simulink model "RobustFormationControl_IntegerModel"  (R2023a)
settings: Solver=ode3  StartTime=0.0  StopTime=30  FixedStep=0.0001  RelTol=1e-3
InitFcn:
  | % % Parameters for the fractional order NTFSMC:
  | % Sliding Surface " Sx, Sy, and Sz ":
  | %------------------------
  | % 10
  | % 10
  | cx = 2*[4 4 4];
  | cxx = 1*[0.01 0.01 0.01];
  | 
  | cx1 = cx(1);
  | cy1 = cx(2);
  | cz1 = cx(3);
  | 
  | cx2 = cxx(1);
  | cy2 = cxx(2);
  | cz2 = cxx(3);
  | 
  | alpha1 = [0.6 0.6 0.6];
  | alpha2 = [0.1 0.1 0.1];
  | 
  | gammaX = [3 3 3];
  | gx  = gammaX(1);
  | gy = gammaX(2);
  | gz = gammaX(3);
  | 
  | p = 10;
  | q = 10;
  | 
  | % Sliding Surface " S_Phi , S_Theta, and  S_Psi":
  | %------------------------
  | cP = 2*[4 4 4];
  | cPP = 1*[0.01 0.01 0.01 0.01];
  | 
  | cPhi1 = cP(1);
  | cTheta1 = cP(2);
  | cPsi1 = cP(3);
  | 
  | cPhi2 = cPP(1);
  | cTheta2 = cPP(2);
  | cPsi2 = cPP(3);
  | gammaP = [3 3 3];
  | 
  | %=========================
  | %=========================
  | SigmaX = 1*[0.01 0.01 0.01];
  | SigmaXX =1*[1 1 1];
  | 
  | Sigma1X = SigmaX(1);
  | Sigma1Y = SigmaX(2);
  | Sigma1Z = SigmaX(3);
  | %-----
  | Sigma2X = SigmaXX(1);
  | Sigma2Y = SigmaXX(2);
  | Sigma2Z = SigmaXX(3);
  | 
  | 
  | SigmaP = 1*[0.01 0.01 0.01];
  | SigmaPP =1*[1 1 1];
  | 
  | Sigma1Phi   = SigmaP(1);
  | Sigma1Theta = SigmaP(2);
  | Sigma1Psi   = SigmaP(3);
  | %----
  | Sigma2Phi   = SigmaPP(1);
  | Sigma2Theta = SigmaPP(2);
  | Sigma2Psi   = SigmaPP(3);
  | 
  | q0 = 0.01;
  | q1 = 0.01;
  | q2 = 0.01;
  | w = 0;
  | %=========================================
  | %=========================================
  | %=========================================
  | %=========================================
  | %=========================================
  | %=========================================
  | %=========================================
  | %=========================================
  | 
  | cxF = 0.01*[4 4 4];
  | cxxF = 1*[0.01 0.01 0.01];
  | 
  | cxF1 = cxF(1);
  | cyF1 = cxF(2);
  | czF1 = cxF(3);
  | 
  | cxF2 = cxxF(1);
  | cyF2 = cxxF(2);
  | czF2 = cxxF(3);
  | 
  | alphaF1 = [0.9 0.9 0.9];
  | alphaF2 = [0.1 0.1 0.1];
  | 
  | gammaX_F = 1.5*[1 1 1];
  | gxF  = gammaX_F(1);
  | gyF = gammaX_F(2);
  | gzF = gammaX_F(3);
  | 
  | % Sliding Surface " S_Phi , S_Theta, and  S_Psi":
  | %------------------------
  | cPF = 1*[4 4 4];
  | cPPF = 1*[0.01 0.01 0.01 0.01];
  | 
  | cPhiF1 = cPF(1);
  | cThetaF1 = cPF(2);
  | cPsiF1 = cPF(3);
  | 
  | cPhiF2 = cPPF(1);
  | cThetaF2 = cPPF(2);
  | cPsiF2 = cPPF(3);
  | gammaP_F = [1 1 1];
  | 
  | %=========================
  | %=========================
  | SigmaXF = 1000*[0.01 0.01 0.01];
  | SigmaXXF =10*[1 1 1];
  | 
  | Sigma1XF = SigmaXF(1);
  | Sigma1YF = SigmaXF(2);
  | Sigma1ZF = SigmaXF(3);
  | %-----
  | Sigma2XF = SigmaXXF(1);
  | Sigma2YF = SigmaXXF(2);
  | Sigma2ZF = SigmaXXF(3);
  | 
  | 
  | SigmaPF = [0.01 0.01 0.01];
  | SigmaPPF =[1 1 1];
  | 
  | Sigma1PhiF   = SigmaPF(1);
  | Sigma1ThetaF = SigmaPF(2);
  | Sigma1PsiF   = SigmaPF(3);
  | %----
  | Sigma2PhiF   = SigmaPPF(1);
  | Sigma2ThetaF = SigmaPPF(2);
  | Sigma2PsiF   = SigmaPPF(3);
  | 
  | % Gain for Exteral Disturbance
  | Dis = 0;
  | dis = 0;
values from neighbouring files (symbols this model uses):
  a1 = (Iyy - Izz)/Ixx    (= -0.812397034596)    [init_quadrotor_params.m]
  a2 = (Izz - Ixx)/Iyy    (= 0.812397034596)    [init_quadrotor_params.m]
  a3 = (Ixx - Iyy)/Izz    (= 0)    [init_quadrotor_params.m]
  a4 = - Ktx/m    (= -0.00114547325103)    [init_quadrotor_params.m]
  a5 = - Kty/m    (= -0.00114547325103)    [init_quadrotor_params.m]
  a6 = - Ktz/m    (= -0.00130740740741)    [init_quadrotor_params.m]
  b = 2.980e-5    (= 2.98e-05)    [init_quadrotor_params.m]
  b1 = - Jr/Ixx    (= -0.00584534596376)    [init_quadrotor_params.m]
  b2 = Jr/Iyy    (= 0.00584534596376)    [init_quadrotor_params.m]
  b3 = - Kfz/Izz    (= -0.0721963413248)    [init_quadrotor_params.m]
  b4 = 1/m    (= 2.05761316872)    [init_quadrotor_params.m]
  b5 = 1/m    (= 2.05761316872)    [init_quadrotor_params.m]
  b6 = 1/m    (= 2.05761316872)    [init_quadrotor_params.m]
  c1 = - Kfx/Ixx    (= -0.114641680395)    [init_quadrotor_params.m]
  c2 = - Kfy/Iyy    (= -0.114641680395)    [init_quadrotor_params.m]
  c3 = 1/Izz    (= 113.62345188)    [init_quadrotor_params.m]
  d = 1.12e-06    [init_quadrotor_params.m]
  d1 = L/Ixx    (= 46.334431631)    [init_quadrotor_params.m]
  d2 = L/Iyy    (= 46.334431631)    [init_quadrotor_params.m]
  g = 9.81    [init_quadrotor_params.m]
  Ixx = 4.856e-3    (= 0.004856)    [init_quadrotor_params.m]
  Iyy = 4.856e-3    (= 0.004856)    [init_quadrotor_params.m]
  Izz = 8.801e-3    (= 0.008801)    [init_quadrotor_params.m]
  Jr = 2.8385e-5    (= 2.8385e-05)    [init_quadrotor_params.m]
  Kfx = 5.567e-4    (= 0.0005567)    [init_quadrotor_params.m]
  Kfy = 5.567e-4    (= 0.0005567)    [init_quadrotor_params.m]
  Kfz = 6.354e-4    (= 0.0006354)    [init_quadrotor_params.m]
  Ktx = 5.5670e-4    (= 0.0005567)    [init_quadrotor_params.m]
  Kty = 5.5670e-4    (= 0.0005567)    [init_quadrotor_params.m]
  Ktz = 6.3540e-4    (= 0.0006354)    [init_quadrotor_params.m]
  L = 0.225    [init_quadrotor_params.m]
  m = 0.486    [init_quadrotor_params.m]
libraries: fod x120, eeStairGenerator x5
(part 1 of 9)
settings Model: Creator=jofan  LastModifiedBy=jofan
settings DataIOCC: ReturnWorkspaceOutputs=off

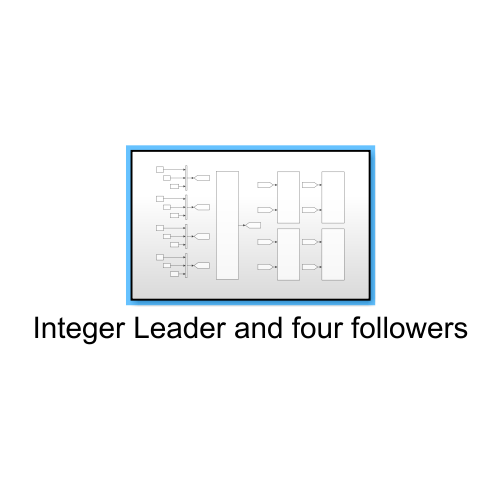
[thumbnail: Simulink's stored preview of the top-level diagram]
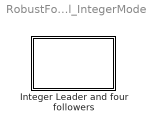
== system RobustFormationControl_IntegerModel ==
  Integer Leader and four followers : Subsystem

== system RobustFormationControl_IntegerModel/Integer Leader and four followers ==
  Follower 1 System : Subsystem
  Follower 2 System : Subsystem
  Follower 3 System : Subsystem
  Follower 4 System : Subsystem
  Leader System : Subsystem
  Mux{,1..3} (4 alike) : Mux  Inputs=3
  dX : Constant  Value=-2
  dX1 : Constant  Value=-2
  dX2 : Constant  Value=-4
  dX3 : Constant  Value=-4
  dY : Constant  Value=2
  dY1 : Constant  Value=-2
  dY2 : Constant  Value=4
  dY3 : Constant  Value=-4
  dZ{,1..3} (4 alike) : Constant  Value=0
  wires:
  dY/1 -> Mux/2
  dZ/1 -> Mux/3
  dX/1 -> Mux/1
  dY1/1 -> Mux1/2
  dZ1/1 -> Mux1/3
  dX1/1 -> Mux1/1
  dX2/1 -> Mux2/1
  dZ2/1 -> Mux2/3
  dY2/1 -> Mux2/2
  dY3/1 -> Mux3/2
  dZ3/1 -> Mux3/3
  dX3/1 -> Mux3/1
  Mux/1 -> [dXYZ]
  Mux1/1 -> [dXYZ1]
  Mux2/1 -> [dXYZ2]
  Mux3/1 -> [dXYZ3]
  Leader System/1(xLeader) -> [xyzL]
  [xyzL] -> Follower 1 System/1(xLeader)
  [xyzL] -> Follower 2 System/1(xLeader)
  [xyzL] -> Follower 4 System/1(xLeader)
  [xyzL] -> Follower 3 System/1(xLeader)
  [dXYZ] -> Follower 1 System/2(dXYZ)
  [dXYZ2] -> Follower 3 System/2(dXYZ)
  [dXYZ1] -> Follower 2 System/2(dXYZ)
  [dXYZ3] -> Follower 4 System/2(dXYZ)

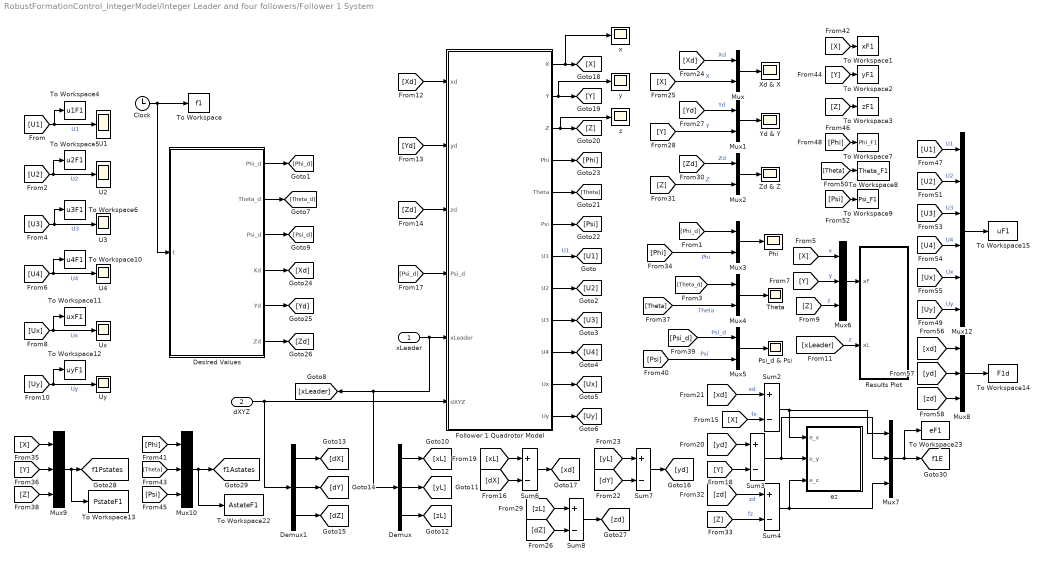
== system RobustFormationControl_IntegerModel/Integer Leader and four followers/Follower 1 System ==
  xLeader : Inport
  dXYZ : Inport  Port=2
  " Phi " : Scope
  Clock : Clock
  Demux : Demux  Outputs=3
  Demux1 : Demux  Outputs=3
  Desired Values : Subsystem
  Follower 1 Quadrotor Model : Subsystem
  Mux{,1..5} (6 alike) : Mux  Inputs=2
  Mux{6..10} (5 alike) : Mux  Inputs=3
  Mux12 : Mux  Inputs=6
  Psi_d & Psi : Scope
  Results Plot : Subsystem
  Sum{2..4,6..8} (6 alike) : Sum  Inputs=+-
  "Theta " : Scope
  To Workspace : ToWorkspace  VariableName=f1  SampleTime=0.03
  To Workspace1 : ToWorkspace  VariableName=xF1  SampleTime=0.03
  To Workspace10 : ToWorkspace  VariableName=u4F1  SampleTime=0.03
  To Workspace11 : ToWorkspace  VariableName=uxF1  SampleTime=0.03
  To Workspace12 : ToWorkspace  VariableName=uyF1  SampleTime=0.03
  To Workspace13 : ToWorkspace  VariableName=PstateF1  SampleTime=-1
  To Workspace14 : ToWorkspace  VariableName=F1d  SampleTime=-1
  To Workspace15 : ToWorkspace  VariableName=uF1  SampleTime=-1
  To Workspace2 : ToWorkspace  VariableName=yF1  SampleTime=0.03
  To Workspace22 : ToWorkspace  VariableName=AstateF1  SampleTime=-1
  To Workspace23 : ToWorkspace  VariableName=eF1  SampleTime=-1
  To Workspace3 : ToWorkspace  VariableName=zF1  SampleTime=0.03
  To Workspace4 : ToWorkspace  VariableName=u1F1  SampleTime=0.03
  To Workspace5 : ToWorkspace  VariableName=u2F1  SampleTime=0.03
  To Workspace6 : ToWorkspace  VariableName=u3F1  SampleTime=0.03
  To Workspace7 : ToWorkspace  VariableName=Phi_F1  SampleTime=0.03
  To Workspace8 : ToWorkspace  VariableName=Theta_F1  SampleTime=0.03
  To Workspace9 : ToWorkspace  VariableName=Psi_F1  SampleTime=0.03
  "U1 " : Scope
  U2 : Scope
  "U3 " : Scope
  "U4 " : Scope
  Ux : Scope
  Uy : Scope
  "Xd & X " : Scope
  Yd & Y : Scope
  "Zd & Z " : Scope
  ez : Subsystem
  x : Scope
  y : Scope
  z : Scope
  tag scope: f1Astates=global, f1E=global, f1Pstates=global
  wires:
  Mux4/1 -> "Theta "/1
  [U2] -> To Workspace5/1, U2/1  "U2"
  [Yd] -> Mux1/1  "Yd"
  Follower 1 Quadrotor Model/10(U4) -> [U4]
  [Zd] -> Follower 1 Quadrotor Model/3(zd)
  [U4] -> To Workspace10/1, "U4 "/1  "U4"
  [Psi] -> To Workspace9/1
  [Z] -> Mux2/2  "Z"
  Follower 1 Quadrotor Model/2(Y) -> y/1, [Y]
  Clock/1 -> To Workspace/1, Desired Values/1(t)
  Follower 1 Quadrotor Model/7(U1) -> [U1]  "U1"
  Desired Values/2(Theta_d) -> [Theta_d]
  Mux2/1 -> "Zd & Z "/1
  [Theta] -> To Workspace8/1
  [Xd] -> Mux/1  "Xd"
  Follower 1 Quadrotor Model/12(Uy) -> [Uy]
  [Y] -> To Workspace2/1
  Follower 1 Quadrotor Model/11(Ux) -> [Ux]
  [X] -> To Workspace1/1
  [Yd] -> Follower 1 Quadrotor Model/2(yd)
  Mux/1 -> "Xd & X "/1
  Follower 1 Quadrotor Model/1(X) -> x/1, [X]
  Mux3/1 -> " Phi "/1
  Follower 1 Quadrotor Model/5(Theta) -> [Theta]
  Mux5/1 -> Psi_d & Psi/1
  [X] -> Mux/2  "X"
  Follower 1 Quadrotor Model/9(U3) -> [U3]
  [Theta] -> Mux4/2  "Theta"
  [Y] -> Mux1/2  "Y"
  [Uy] -> To Workspace12/1, Uy/1  "Uy"
  Desired Values/3(Psi_d) -> [Psi_d]
  Follower 1 Quadrotor Model/3(Z) -> z/1, [Z]
  [U1] -> To Workspace4/1, "U1 "/1  "U1"
  [Ux] -> To Workspace11/1, Ux/1  "Ux"
  Desired Values/6(Zd) -> [Zd]
  [Phi] -> Mux3/2  "Phi"
  Mux1/1 -> Yd & Y/1
  [Xd] -> Follower 1 Quadrotor Model/1(xd)
  [Psi] -> Mux5/2  "Psi"
  [Z] -> To Workspace3/1
  Follower 1 Quadrotor Model/8(U2) -> [U2]
  [Theta_d] -> Mux4/1
  [Psi_d] -> Mux5/1  "Psi_d"
  [Zd] -> Mux2/1  "Zd"
  [U3] -> To Workspace6/1, "U3 "/1  "U3"
  Desired Values/5(Yd) -> [Yd]
  [Psi_d] -> Follower 1 Quadrotor Model/4(Psi_d)
  Follower 1 Quadrotor Model/6(Psi) -> [Psi]
  Follower 1 Quadrotor Model/4(Phi) -> [Phi]
  Desired Values/4(Xd) -> [Xd]
  [Phi_d] -> Mux3/1
  Desired Values/1(Phi_d) -> [Phi_d]
  [Phi] -> To Workspace7/1
  [Z] -> Mux6/3  "z"
  [X] -> Mux6/1  "x"
  [xLeader] -> Results Plot/2(xL)  "z"
  Mux6/1 -> Results Plot/1(xF)
  [Y] -> Mux6/2  "y"
  Sum7/1 -> [yd]
  [dY] -> Sum7/2
  [yL] -> Sum7/1
  Demux/3 -> [zL]
  xLeader/1 -> [xLeader], Demux/1, Follower 1 Quadrotor Model/5(xLeader)
  Demux1/1 -> [dX]
  [zd] -> Sum4/1  "zd"
  Demux/1 -> [xL]
  [X] -> Sum2/2  "fx"
  dXYZ/1 -> Demux1/1, Follower 1 Quadrotor Model/6(dXYZ)
  Demux1/2 -> [dY]
  [xL] -> Sum6/1
  Sum4/1 -> Mux7/3, ez/3(e_z)
  Sum3/1 -> Mux7/2, ez/2(e_y)
  Sum2/1 -> Mux7/1, ez/1(e_x)
  [dZ] -> Sum8/2
  [Z] -> Sum4/2  "fz"
  Demux/2 -> [yL]
  [dX] -> Sum6/2
  [yd] -> Sum3/1
  [Y] -> Sum3/2
  [xd] -> Sum2/1  "xd"
  Sum8/1 -> [zd]
  Demux1/3 -> [dZ]
  [zL] -> Sum8/1
  Sum6/1 -> [xd]
  Mux10/1 -> To Workspace22/1, [f1Astates]
  [Psi] -> Mux10/3
  [Phi] -> Mux10/1
  Mux9/1 -> To Workspace13/1, [f1Pstates]
  [Z] -> Mux9/3
  [Y] -> Mux9/2
  [X] -> Mux9/1
  [Theta] -> Mux10/2
  Mux7/1 -> To Workspace23/1, [f1E]
  [Ux] -> Mux12/5  "Ux"
  [U3] -> Mux12/3  "U3"
  [U2] -> Mux12/2  "U2"
  [U4] -> Mux12/4  "U4"
  [Uy] -> Mux12/6  "Uy"
  [U1] -> Mux12/1  "U1"
  Mux8/1 -> To Workspace14/1
  [xd] -> Mux8/1
  [yd] -> Mux8/2
  [zd] -> Mux8/3
  Mux12/1 -> To Workspace15/1

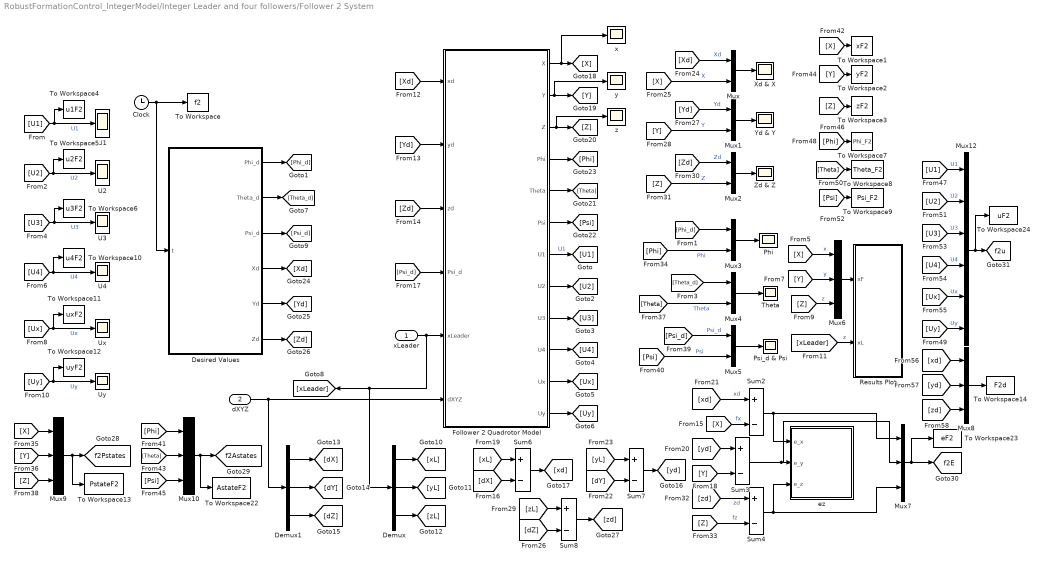
== system RobustFormationControl_IntegerModel/Integer Leader and four followers/Follower 2 System ==
  xLeader : Inport
  dXYZ : Inport  Port=2
  " Phi " : Scope
  Clock : Clock
  Demux : Demux  Outputs=3
  Demux1 : Demux  Outputs=3
  Desired Values : Subsystem
  Follower 2 Quadrotor Model : Subsystem
  Mux{,1..5} (6 alike) : Mux  Inputs=2
  Mux{6..10} (5 alike) : Mux  Inputs=3
  Mux12 : Mux  Inputs=6
  Psi_d & Psi : Scope
  Results Plot : Subsystem
  Sum{2..4,6..8} (6 alike) : Sum  Inputs=+-
  "Theta " : Scope
  To Workspace : ToWorkspace  VariableName=f2  SampleTime=0.03
  To Workspace1 : ToWorkspace  VariableName=xF2  SampleTime=0.03
  To Workspace10 : ToWorkspace  VariableName=u4F2  SampleTime=0.03
  To Workspace11 : ToWorkspace  VariableName=uxF2  SampleTime=0.03
  To Workspace12 : ToWorkspace  VariableName=uyF2  SampleTime=0.03
  To Workspace13 : ToWorkspace  VariableName=PstateF2  SampleTime=-1
  To Workspace14 : ToWorkspace  VariableName=F2d  SampleTime=-1
  To Workspace2 : ToWorkspace  VariableName=yF2  SampleTime=0.03
  To Workspace22 : ToWorkspace  VariableName=AstateF2  SampleTime=-1
  To Workspace23 : ToWorkspace  VariableName=eF2  SampleTime=-1
  To Workspace24 : ToWorkspace  VariableName=uF2  SampleTime=-1
  To Workspace3 : ToWorkspace  VariableName=zF2  SampleTime=0.03
  To Workspace4 : ToWorkspace  VariableName=u1F2  SampleTime=0.03
  To Workspace5 : ToWorkspace  VariableName=u2F2  SampleTime=0.03
  To Workspace6 : ToWorkspace  VariableName=u3F2  SampleTime=0.03
  To Workspace7 : ToWorkspace  VariableName=Phi_F2  SampleTime=0.03
  To Workspace8 : ToWorkspace  VariableName=Theta_F2  SampleTime=0.03
  To Workspace9 : ToWorkspace  VariableName=Psi_F2  SampleTime=0.03
  "U1 " : Scope
  U2 : Scope
  "U3 " : Scope
  "U4 " : Scope
  Ux : Scope
  Uy : Scope
  "Xd & X " : Scope
  Yd & Y : Scope
  "Zd & Z " : Scope
  ez : Subsystem
  x : Scope
  y : Scope
  z : Scope
  tag scope: f2Astates=global, f2E=global, f2Pstates=global, f2u=global
  wires:
  Mux4/1 -> "Theta "/1
  [U2] -> To Workspace5/1, U2/1  "U2"
  [Yd] -> Mux1/1  "Yd"
  Follower 2 Quadrotor Model/10(U4) -> [U4]
  [Zd] -> Follower 2 Quadrotor Model/3(zd)
  [U4] -> To Workspace10/1, "U4 "/1  "U4"
  [Psi] -> To Workspace9/1
  [Z] -> Mux2/2  "Z"
  Follower 2 Quadrotor Model/2(Y) -> y/1, [Y]
  Clock/1 -> To Workspace/1, Desired Values/1(t)
  Follower 2 Quadrotor Model/7(U1) -> [U1]  "U1"
  Desired Values/2(Theta_d) -> [Theta_d]
  Mux2/1 -> "Zd & Z "/1
  [Theta] -> To Workspace8/1
  [Xd] -> Mux/1  "Xd"
  Follower 2 Quadrotor Model/12(Uy) -> [Uy]
  [Y] -> To Workspace2/1
  Follower 2 Quadrotor Model/11(Ux) -> [Ux]
  [X] -> To Workspace1/1
  [Yd] -> Follower 2 Quadrotor Model/2(yd)
  Mux/1 -> "Xd & X "/1
  Follower 2 Quadrotor Model/1(X) -> x/1, [X]
  Mux3/1 -> " Phi "/1
  Follower 2 Quadrotor Model/5(Theta) -> [Theta]
  Mux5/1 -> Psi_d & Psi/1
  [X] -> Mux/2  "X"
  Follower 2 Quadrotor Model/9(U3) -> [U3]
  [Theta] -> Mux4/2  "Theta"
  [Y] -> Mux1/2  "Y"
  [Uy] -> To Workspace12/1, Uy/1  "Uy"
  Desired Values/3(Psi_d) -> [Psi_d]
  Follower 2 Quadrotor Model/3(Z) -> z/1, [Z]
  [U1] -> To Workspace4/1, "U1 "/1  "U1"
  [Ux] -> To Workspace11/1, Ux/1  "Ux"
  Desired Values/6(Zd) -> [Zd]
  [Phi] -> Mux3/2  "Phi"
  Mux1/1 -> Yd & Y/1
  [Xd] -> Follower 2 Quadrotor Model/1(xd)
  [Psi] -> Mux5/2  "Psi"
  [Z] -> To Workspace3/1
  Follower 2 Quadrotor Model/8(U2) -> [U2]
  [Theta_d] -> Mux4/1
  [Psi_d] -> Mux5/1  "Psi_d"
  [Zd] -> Mux2/1  "Zd"
  [U3] -> To Workspace6/1, "U3 "/1  "U3"
  Desired Values/5(Yd) -> [Yd]
  [Psi_d] -> Follower 2 Quadrotor Model/4(Psi_d)
  Follower 2 Quadrotor Model/6(Psi) -> [Psi]
  Follower 2 Quadrotor Model/4(Phi) -> [Phi]
  Desired Values/4(Xd) -> [Xd]
  [Phi_d] -> Mux3/1
  Desired Values/1(Phi_d) -> [Phi_d]
  [Phi] -> To Workspace7/1
  xLeader/1 -> Demux/1, [xLeader], Follower 2 Quadrotor Model/5(xLeader)
  [Z] -> Mux6/3  "z"
  [X] -> Mux6/1  "x"
  [xLeader] -> Results Plot/2(xL)  "z"
  Mux6/1 -> Results Plot/1(xF)
  [Y] -> Mux6/2  "y"
  Sum7/1 -> [yd]
  [dY] -> Sum7/2
  [yL] -> Sum7/1
  Demux/3 -> [zL]
  Demux1/1 -> [dX]
  [zd] -> Sum4/1  "zd"
  Demux/1 -> [xL]
  [X] -> Sum2/2  "fx"
  dXYZ/1 -> Demux1/1, Follower 2 Quadrotor Model/6(dXYZ)
  Demux1/2 -> [dY]
  [xL] -> Sum6/1
  Sum4/1 -> Mux7/3, ez/3(e_z)
  Sum3/1 -> Mux7/2, ez/2(e_y)
  Sum2/1 -> Mux7/1, ez/1(e_x)
  [dZ] -> Sum8/2
  [Z] -> Sum4/2  "fz"
  Demux/2 -> [yL]
  [dX] -> Sum6/2
  [yd] -> Sum3/1
  [Y] -> Sum3/2
  [xd] -> Sum2/1  "xd"
  Sum8/1 -> [zd]
  Demux1/3 -> [dZ]
  [zL] -> Sum8/1
  Sum6/1 -> [xd]
  [X] -> Mux9/1
  [Psi] -> Mux10/3
  [Theta] -> Mux10/2
  Mux9/1 -> To Workspace13/1, [f2Pstates]
  [Y] -> Mux9/2
  [Phi] -> Mux10/1
  Mux10/1 -> To Workspace22/1, [f2Astates]
  [Z] -> Mux9/3
  Mux7/1 -> To Workspace23/1, [f2E]
  [U3] -> Mux12/3  "U3"
  [Ux] -> Mux12/5  "Ux"
  Mux12/1 -> To Workspace24/1, [f2u]
  [Uy] -> Mux12/6  "Uy"
  [U4] -> Mux12/4  "U4"
  [U2] -> Mux12/2  "U2"
  [U1] -> Mux12/1  "U1"
  Mux8/1 -> To Workspace14/1
  [zd] -> Mux8/3
  [xd] -> Mux8/1
  [yd] -> Mux8/2

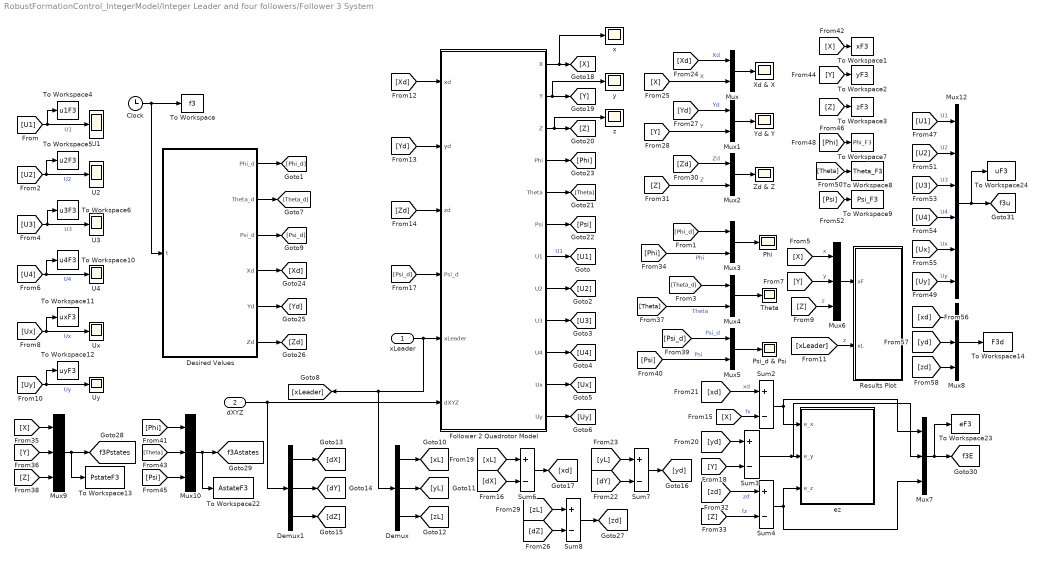
== system RobustFormationControl_IntegerModel/Integer Leader and four followers/Follower 3 System ==
  xLeader : Inport
  dXYZ : Inport  Port=2
  " Phi " : Scope
  Clock : Clock
  Demux : Demux  Outputs=3
  Demux1 : Demux  Outputs=3
  Desired Values : Subsystem
  Follower 2 Quadrotor Model : Subsystem
  Mux{,1..5} (6 alike) : Mux  Inputs=2
  Mux{6..10} (5 alike) : Mux  Inputs=3
  Mux12 : Mux  Inputs=6
  Psi_d & Psi : Scope
  Results Plot : Subsystem
  Sum{2..4,6..8} (6 alike) : Sum  Inputs=+-
  "Theta " : Scope
  To Workspace : ToWorkspace  VariableName=f3  SampleTime=0.03
  To Workspace1 : ToWorkspace  VariableName=xF3  SampleTime=0.03
  To Workspace10 : ToWorkspace  VariableName=u4F3  SampleTime=0.03
  To Workspace11 : ToWorkspace  VariableName=uxF3  SampleTime=0.03
  To Workspace12 : ToWorkspace  VariableName=uyF3  SampleTime=0.03
  To Workspace13 : ToWorkspace  VariableName=PstateF3  SampleTime=-1
  To Workspace14 : ToWorkspace  VariableName=F3d  SampleTime=-1
  To Workspace2 : ToWorkspace  VariableName=yF3  SampleTime=0.03
  To Workspace22 : ToWorkspace  VariableName=AstateF3  SampleTime=-1
  To Workspace23 : ToWorkspace  VariableName=eF3  SampleTime=-1
  To Workspace24 : ToWorkspace  VariableName=uF3  SampleTime=-1
  To Workspace3 : ToWorkspace  VariableName=zF3  SampleTime=0.03
  To Workspace4 : ToWorkspace  VariableName=u1F3  SampleTime=0.03
  To Workspace5 : ToWorkspace  VariableName=u2F3  SampleTime=0.03
  To Workspace6 : ToWorkspace  VariableName=u3F3  SampleTime=0.03
  To Workspace7 : ToWorkspace  VariableName=Phi_F3  SampleTime=0.03
  To Workspace8 : ToWorkspace  VariableName=Theta_F3  SampleTime=0.03
  To Workspace9 : ToWorkspace  VariableName=Psi_F3  SampleTime=0.03
  "U1 " : Scope
  U2 : Scope
  "U3 " : Scope
  "U4 " : Scope
  Ux : Scope
  Uy : Scope
  "Xd & X " : Scope
  Yd & Y : Scope
  "Zd & Z " : Scope
  ez : Subsystem
  x : Scope
  y : Scope
  z : Scope
  tag scope: f3Astates=global, f3E=global, f3Pstates=global, f3u=global
  wires:
  [Y] -> Mux6/2  "y"
  Mux6/1 -> Results Plot/1(xF)
  [xLeader] -> Results Plot/2(xL)  "z"
  [X] -> Mux6/1  "x"
  [Z] -> Mux6/3  "z"
  xLeader/1 -> Follower 2 Quadrotor Model/5(xLeader), Demux/1, [xLeader]
  [Phi] -> To Workspace7/1
  Desired Values/1(Phi_d) -> [Phi_d]
  [Phi_d] -> Mux3/1
  Desired Values/4(Xd) -> [Xd]
  Follower 2 Quadrotor Model/4(Phi) -> [Phi]
  Follower 2 Quadrotor Model/6(Psi) -> [Psi]
  [Psi_d] -> Follower 2 Quadrotor Model/4(Psi_d)
  Desired Values/5(Yd) -> [Yd]
  [U3] -> "U3 "/1, To Workspace6/1  "U3"
  [Zd] -> Mux2/1  "Zd"
  [Psi_d] -> Mux5/1  "Psi_d"
  [Theta_d] -> Mux4/1
  Follower 2 Quadrotor Model/8(U2) -> [U2]
  [Z] -> To Workspace3/1
  [Psi] -> Mux5/2  "Psi"
  [Xd] -> Follower 2 Quadrotor Model/1(xd)
  Mux1/1 -> Yd & Y/1
  [Phi] -> Mux3/2  "Phi"
  Desired Values/6(Zd) -> [Zd]
  [Ux] -> Ux/1, To Workspace11/1  "Ux"
  [U1] -> "U1 "/1, To Workspace4/1  "U1"
  Follower 2 Quadrotor Model/3(Z) -> [Z], z/1
  Desired Values/3(Psi_d) -> [Psi_d]
  [Uy] -> Uy/1, To Workspace12/1  "Uy"
  [Y] -> Mux1/2  "Y"
  [Theta] -> Mux4/2  "Theta"
  Follower 2 Quadrotor Model/9(U3) -> [U3]
  [X] -> Mux/2  "X"
  Mux5/1 -> Psi_d & Psi/1
  Follower 2 Quadrotor Model/5(Theta) -> [Theta]
  Mux3/1 -> " Phi "/1
  Follower 2 Quadrotor Model/1(X) -> [X], x/1
  Mux/1 -> "Xd & X "/1
  [Yd] -> Follower 2 Quadrotor Model/2(yd)
  [X] -> To Workspace1/1
  Follower 2 Quadrotor Model/11(Ux) -> [Ux]
  [Y] -> To Workspace2/1
  Follower 2 Quadrotor Model/12(Uy) -> [Uy]
  [Xd] -> Mux/1  "Xd"
  [Theta] -> To Workspace8/1
  Mux2/1 -> "Zd & Z "/1
  Desired Values/2(Theta_d) -> [Theta_d]
  Follower 2 Quadrotor Model/7(U1) -> [U1]  "U1"
  Clock/1 -> Desired Values/1(t), To Workspace/1
  Follower 2 Quadrotor Model/2(Y) -> [Y], y/1
  [Z] -> Mux2/2  "Z"
  [Psi] -> To Workspace9/1
  [U4] -> "U4 "/1, To Workspace10/1  "U4"
  [Zd] -> Follower 2 Quadrotor Model/3(zd)
  Follower 2 Quadrotor Model/10(U4) -> [U4]
  [Yd] -> Mux1/1  "Yd"
  [U2] -> U2/1, To Workspace5/1  "U2"
  Mux4/1 -> "Theta "/1
  Sum7/1 -> [yd]
  [dY] -> Sum7/2
  [yL] -> Sum7/1
  Demux/3 -> [zL]
  Demux1/1 -> [dX]
  [zd] -> Sum4/1  "zd"
  Demux/1 -> [xL]
  [X] -> Sum2/2  "fx"
  dXYZ/1 -> Demux1/1, Follower 2 Quadrotor Model/6(dXYZ)
  Demux1/2 -> [dY]
  [xL] -> Sum6/1
  Sum4/1 -> Mux7/3, ez/3(e_z)
  Sum3/1 -> Mux7/2, ez/2(e_y)
  Sum2/1 -> Mux7/1, ez/1(e_x)
  [dZ] -> Sum8/2
  [Z] -> Sum4/2  "fz"
  Demux/2 -> [yL]
  [dX] -> Sum6/2
  [yd] -> Sum3/1
  [Y] -> Sum3/2
  [xd] -> Sum2/1  "xd"
  Sum8/1 -> [zd]
  Demux1/3 -> [dZ]
  [zL] -> Sum8/1
  Sum6/1 -> [xd]
  [X] -> Mux9/1
  [Psi] -> Mux10/3
  [Theta] -> Mux10/2
  Mux9/1 -> To Workspace13/1, [f3Pstates]
  [Y] -> Mux9/2
  [Phi] -> Mux10/1
  Mux10/1 -> To Workspace22/1, [f3Astates]
  [Z] -> Mux9/3
  Mux7/1 -> To Workspace23/1, [f3E]
  [U3] -> Mux12/3  "U3"
  [Ux] -> Mux12/5  "Ux"
  Mux12/1 -> To Workspace24/1, [f3u]
  [Uy] -> Mux12/6  "Uy"
  [U4] -> Mux12/4  "U4"
  [U2] -> Mux12/2  "U2"
  [U1] -> Mux12/1  "U1"
  Mux8/1 -> To Workspace14/1
  [zd] -> Mux8/3
  [xd] -> Mux8/1
  [yd] -> Mux8/2

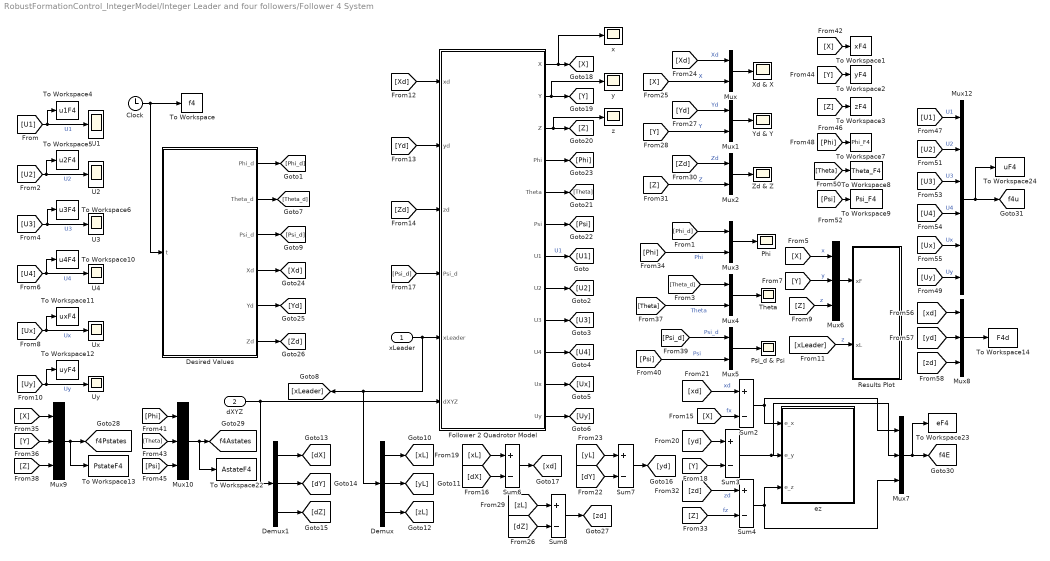
== system RobustFormationControl_IntegerModel/Integer Leader and four followers/Follower 4 System ==
  xLeader : Inport
  dXYZ : Inport  Port=2
  " Phi " : Scope
  Clock : Clock
  Demux : Demux  Outputs=3
  Demux1 : Demux  Outputs=3
  Desired Values : Subsystem
  Follower 2 Quadrotor Model : Subsystem
  Mux{,1..5} (6 alike) : Mux  Inputs=2
  Mux{6..10} (5 alike) : Mux  Inputs=3
  Mux12 : Mux  Inputs=6
  Psi_d & Psi : Scope
  Results Plot : Subsystem
  Sum{2..4,6..8} (6 alike) : Sum  Inputs=+-
  "Theta " : Scope
  To Workspace : ToWorkspace  VariableName=f4  SampleTime=0.03
  To Workspace1 : ToWorkspace  VariableName=xF4  SampleTime=0.03
  To Workspace10 : ToWorkspace  VariableName=u4F4  SampleTime=0.03
  To Workspace11 : ToWorkspace  VariableName=uxF4  SampleTime=0.03
  To Workspace12 : ToWorkspace  VariableName=uyF4  SampleTime=0.03
  To Workspace13 : ToWorkspace  VariableName=PstateF4  SampleTime=-1
  To Workspace14 : ToWorkspace  VariableName=F4d  SampleTime=-1
  To Workspace2 : ToWorkspace  VariableName=yF4  SampleTime=0.03
  To Workspace22 : ToWorkspace  VariableName=AstateF4  SampleTime=-1
  To Workspace23 : ToWorkspace  VariableName=eF4  SampleTime=-1
  To Workspace24 : ToWorkspace  VariableName=uF4  SampleTime=-1
  To Workspace3 : ToWorkspace  VariableName=zF4  SampleTime=0.03
  To Workspace4 : ToWorkspace  VariableName=u1F4  SampleTime=0.03
  To Workspace5 : ToWorkspace  VariableName=u2F4  SampleTime=0.03
  To Workspace6 : ToWorkspace  VariableName=u3F4  SampleTime=0.03
  To Workspace7 : ToWorkspace  VariableName=Phi_F4  SampleTime=0.03
  To Workspace8 : ToWorkspace  VariableName=Theta_F4  SampleTime=0.03
  To Workspace9 : ToWorkspace  VariableName=Psi_F4  SampleTime=0.03
  "U1 " : Scope
  U2 : Scope
  "U3 " : Scope
  "U4 " : Scope
  Ux : Scope
  Uy : Scope
  "Xd & X " : Scope
  Yd & Y : Scope
  "Zd & Z " : Scope
  ez : Subsystem
  x : Scope
  y : Scope
  z : Scope
  tag scope: f4Astates=global, f4E=global, f4Pstates=global, f4u=global
  wires:
  Mux4/1 -> "Theta "/1
  [U2] -> To Workspace5/1, U2/1  "U2"
  [Yd] -> Mux1/1  "Yd"
  Follower 2 Quadrotor Model/10(U4) -> [U4]
  [Zd] -> Follower 2 Quadrotor Model/3(zd)
  [U4] -> To Workspace10/1, "U4 "/1  "U4"
  [Psi] -> To Workspace9/1
  [Z] -> Mux2/2  "Z"
  Follower 2 Quadrotor Model/2(Y) -> y/1, [Y]
  Clock/1 -> To Workspace/1, Desired Values/1(t)
  Follower 2 Quadrotor Model/7(U1) -> [U1]  "U1"
  Desired Values/2(Theta_d) -> [Theta_d]
  Mux2/1 -> "Zd & Z "/1
  [Theta] -> To Workspace8/1
  [Xd] -> Mux/1  "Xd"
  Follower 2 Quadrotor Model/12(Uy) -> [Uy]
  [Y] -> To Workspace2/1
  Follower 2 Quadrotor Model/11(Ux) -> [Ux]
  [X] -> To Workspace1/1
  [Yd] -> Follower 2 Quadrotor Model/2(yd)
  Mux/1 -> "Xd & X "/1
  Follower 2 Quadrotor Model/1(X) -> x/1, [X]
  Mux3/1 -> " Phi "/1
  Follower 2 Quadrotor Model/5(Theta) -> [Theta]
  Mux5/1 -> Psi_d & Psi/1
  [X] -> Mux/2  "X"
  Follower 2 Quadrotor Model/9(U3) -> [U3]
  [Theta] -> Mux4/2  "Theta"
  [Y] -> Mux1/2  "Y"
  [Uy] -> To Workspace12/1, Uy/1  "Uy"
  Desired Values/3(Psi_d) -> [Psi_d]
  Follower 2 Quadrotor Model/3(Z) -> z/1, [Z]
  [U1] -> To Workspace4/1, "U1 "/1  "U1"
  [Ux] -> To Workspace11/1, Ux/1  "Ux"
  Desired Values/6(Zd) -> [Zd]
  [Phi] -> Mux3/2  "Phi"
  Mux1/1 -> Yd & Y/1
  [Xd] -> Follower 2 Quadrotor Model/1(xd)
  [Psi] -> Mux5/2  "Psi"
  [Z] -> To Workspace3/1
  Follower 2 Quadrotor Model/8(U2) -> [U2]
  [Theta_d] -> Mux4/1
  [Psi_d] -> Mux5/1  "Psi_d"
  [Zd] -> Mux2/1  "Zd"
  [U3] -> To Workspace6/1, "U3 "/1  "U3"
  Desired Values/5(Yd) -> [Yd]
  [Psi_d] -> Follower 2 Quadrotor Model/4(Psi_d)
  Follower 2 Quadrotor Model/6(Psi) -> [Psi]
  Follower 2 Quadrotor Model/4(Phi) -> [Phi]
  Desired Values/4(Xd) -> [Xd]
  [Phi_d] -> Mux3/1
  Desired Values/1(Phi_d) -> [Phi_d]
  [Phi] -> To Workspace7/1
  [Z] -> Mux6/3  "z"
  [X] -> Mux6/1  "x"
  [xLeader] -> Results Plot/2(xL)  "z"
  Mux6/1 -> Results Plot/1(xF)
  [Y] -> Mux6/2  "y"
  Sum7/1 -> [yd]
  [dY] -> Sum7/2
  [yL] -> Sum7/1
  Demux/3 -> [zL]
  xLeader/1 -> Demux/1, [xLeader], Follower 2 Quadrotor Model/5(xLeader)
  Demux1/1 -> [dX]
  [zd] -> Sum4/1  "zd"
  Demux/1 -> [xL]
  [X] -> Sum2/2  "fx"
  dXYZ/1 -> Follower 2 Quadrotor Model/6(dXYZ), Demux1/1
  Demux1/2 -> [dY]
  [xL] -> Sum6/1
  Sum4/1 -> Mux7/3, ez/3(e_z)
  Sum3/1 -> Mux7/2, ez/2(e_y)
  Sum2/1 -> Mux7/1, ez/1(e_x)
  [dZ] -> Sum8/2
  [Z] -> Sum4/2  "fz"
  Demux/2 -> [yL]
  [dX] -> Sum6/2
  [yd] -> Sum3/1
  [Y] -> Sum3/2
  [xd] -> Sum2/1  "xd"
  Sum8/1 -> [zd]
  Demux1/3 -> [dZ]
  [zL] -> Sum8/1
  Sum6/1 -> [xd]
  [X] -> Mux9/1
  [Psi] -> Mux10/3
  [Theta] -> Mux10/2
  Mux9/1 -> To Workspace13/1, [f4Pstates]
  [Y] -> Mux9/2
  [Phi] -> Mux10/1
  Mux10/1 -> To Workspace22/1, [f4Astates]
  [Z] -> Mux9/3
  Mux7/1 -> To Workspace23/1, [f4E]
  [U3] -> Mux12/3  "U3"
  [Ux] -> Mux12/5  "Ux"
  Mux12/1 -> To Workspace24/1, [f4u]
  [Uy] -> Mux12/6  "Uy"
  [U4] -> Mux12/4  "U4"
  [U2] -> Mux12/2  "U2"
  [U1] -> Mux12/1  "U1"
  Mux8/1 -> To Workspace14/1
  [zd] -> Mux8/3
  [xd] -> Mux8/1
  [yd] -> Mux8/2

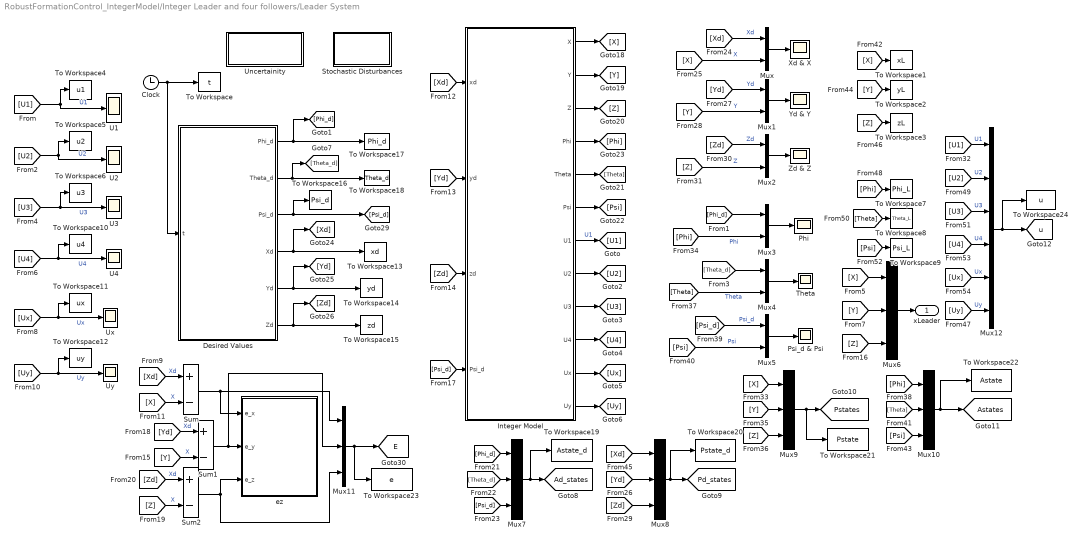
== system RobustFormationControl_IntegerModel/Integer Leader and four followers/Leader System ==
  " Phi " : Scope
  Clock : Clock
  Desired Values : Subsystem
  Integer Model : Subsystem
  Mux{,1..5} (6 alike) : Mux  Inputs=2
  Mux{6..11} (6 alike) : Mux  Inputs=3
  Mux12 : Mux  Inputs=6
  Psi_d & Psi : Scope
  Stochastic Disturbances : Subsystem
  Sum : Sum  Inputs=+-
  Sum1 : Sum  Inputs=+-
  Sum2 : Sum  Inputs=+-
  "Theta " : Scope
  To Workspace : ToWorkspace  VariableName=t  SampleTime=0.03
  To Workspace1 : ToWorkspace  VariableName=xL  SampleTime=0.03
  To Workspace10 : ToWorkspace  VariableName=u4  SampleTime=-1
  To Workspace11 : ToWorkspace  VariableName=ux  SampleTime=0.03
  To Workspace12 : ToWorkspace  VariableName=uy  SampleTime=0.03
  To Workspace13 : ToWorkspace  VariableName=xd  SampleTime=0.03
  To Workspace14 : ToWorkspace  VariableName=yd  SampleTime=0.03
  To Workspace15 : ToWorkspace  VariableName=zd  SampleTime=0.03
  To Workspace16 : ToWorkspace  VariableName=Psi_d  SampleTime=0.03
  To Workspace17 : ToWorkspace  VariableName=Phi_d  SampleTime=0.03
  To Workspace18 : ToWorkspace  VariableName=Theta_d  SampleTime=0.03
  To Workspace19 : ToWorkspace  VariableName=Astate_d  SampleTime=-1
  To Workspace2 : ToWorkspace  VariableName=yL  SampleTime=0.03
  To Workspace20 : ToWorkspace  VariableName=Pstate_d  SampleTime=-1
  To Workspace21 : ToWorkspace  VariableName=Pstate  SampleTime=-1
  To Workspace22 : ToWorkspace  VariableName=Astate  SampleTime=-1
  To Workspace23 : ToWorkspace  VariableName=e  SampleTime=-1
  To Workspace24 : ToWorkspace  VariableName=u  SampleTime=-1
  To Workspace3 : ToWorkspace  VariableName=zL  SampleTime=0.03
  To Workspace4 : ToWorkspace  VariableName=u1  SampleTime=0.03
  To Workspace5 : ToWorkspace  VariableName=u2  SampleTime=0.03
  To Workspace6 : ToWorkspace  VariableName=u3  SampleTime=0.03
  To Workspace7 : ToWorkspace  VariableName=Phi_L  SampleTime=0.03
  To Workspace8 : ToWorkspace  VariableName=Theta_L  SampleTime=0.03
  To Workspace9 : ToWorkspace  VariableName=Psi_L  SampleTime=0.03
  "U1 " : Scope
  U2 : Scope
  "U3 " : Scope
  "U4 " : Scope
  Uncertainity : Subsystem
  Ux : Scope
  Uy : Scope
  "Xd & X " : Scope
  Yd & Y : Scope
  "Zd & Z " : Scope
  ez : Subsystem
  xLeader : Outport
  tag scope: Ad_states=global, Astates=global, E=global, Pd_states=global, Pstates=global, u=global
  wires:
  Mux4/1 -> "Theta "/1
  [U2] -> To Workspace5/1, U2/1  "U2"
  [Yd] -> Mux1/1  "Yd"
  Integer Model/10(U4) -> [U4]
  [Zd] -> Integer Model/3(zd)
  [U4] -> To Workspace10/1, "U4 "/1  "U4"
  [Psi] -> To Workspace9/1
  [Z] -> Mux2/2  "Z"
  Integer Model/2(Y) -> [Y]
  Clock/1 -> To Workspace/1, Desired Values/1(t)
  Integer Model/7(U1) -> [U1]  "U1"
  Desired Values/2(Theta_d) -> To Workspace18/1, [Theta_d]
  Mux2/1 -> "Zd & Z "/1
  [Theta] -> To Workspace8/1
  [Xd] -> Mux/1  "Xd"
  Integer Model/12(Uy) -> [Uy]
  [Y] -> To Workspace2/1
  Integer Model/11(Ux) -> [Ux]
  [X] -> To Workspace1/1
  [Yd] -> Integer Model/2(yd)
  Mux/1 -> "Xd & X "/1
  Integer Model/1(X) -> [X]
  Mux3/1 -> " Phi "/1
  Integer Model/5(Theta) -> [Theta]
  Mux5/1 -> Psi_d & Psi/1
  [X] -> Mux/2  "X"
  Integer Model/9(U3) -> [U3]
  [Theta] -> Mux4/2  "Theta"
  [Y] -> Mux1/2  "Y"
  [Uy] -> To Workspace12/1, Uy/1  "Uy"
  Desired Values/3(Psi_d) -> To Workspace16/1, [Psi_d]
  Integer Model/3(Z) -> [Z]
  [U1] -> To Workspace4/1, "U1 "/1  "U1"
  [Ux] -> To Workspace11/1, Ux/1  "Ux"
  Desired Values/6(Zd) -> [Zd], To Workspace15/1
  [Phi] -> Mux3/2  "Phi"
  Mux1/1 -> Yd & Y/1
  [Xd] -> Integer Model/1(xd)
  [Psi] -> Mux5/2  "Psi"
  [Z] -> To Workspace3/1
  Integer Model/8(U2) -> [U2]
  [Theta_d] -> Mux4/1
  [Psi_d] -> Mux5/1  "Psi_d"
  [Zd] -> Mux2/1  "Zd"
  [U3] -> To Workspace6/1, "U3 "/1  "U3"
  Desired Values/5(Yd) -> [Yd], To Workspace14/1
  [Psi_d] -> Integer Model/4(Psi_d)
  Integer Model/6(Psi) -> [Psi]
  Integer Model/4(Phi) -> [Phi]
  Desired Values/4(Xd) -> [Xd], To Workspace13/1
  [Phi_d] -> Mux3/1
  Desired Values/1(Phi_d) -> To Workspace17/1, [Phi_d]
  [Phi] -> To Workspace7/1
  [X] -> Mux6/1
  Mux6/1 -> xLeader/1
  [Z] -> Mux6/3
  [Y] -> Mux6/2
  [Xd] -> Sum/1  "Xd"
  [X] -> Sum/2  "X"
  [Y] -> Sum1/2  "X"
  [Yd] -> Sum1/1  "Xd"
  [Z] -> Sum2/2  "X"
  [Zd] -> Sum2/1  "Xd"
  Sum1/1 -> Mux11/2, ez/2(e_y)
  Sum/1 -> Mux11/1, ez/1(e_x)
  Sum2/1 -> Mux11/3, ez/3(e_z)
  [Phi_d] -> Mux7/1
  [Theta_d] -> Mux7/2
  [Psi_d] -> Mux7/3
  Mux7/1 -> To Workspace19/1, [Ad_states]
  Mux8/1 -> To Workspace20/1, [Pd_states]
  [Xd] -> Mux8/1
  [Zd] -> Mux8/3
  [Yd] -> Mux8/2
  Mux9/1 -> To Workspace21/1, [Pstates]
  Mux10/1 -> To Workspace22/1, [Astates]
  [Psi] -> Mux10/3
  [Theta] -> Mux10/2
  [X] -> Mux9/1
  [Phi] -> Mux10/1
  [Z] -> Mux9/3
  [Y] -> Mux9/2
  Mux11/1 -> To Workspace23/1, [E]
  Mux12/1 -> To Workspace24/1, [u]
  [U1] -> Mux12/1  "U1"
  [U2] -> Mux12/2  "U2"
  [U3] -> Mux12/3  "U3"
  [U4] -> Mux12/4  "U4"
  [Ux] -> Mux12/5  "Ux"
  [Uy] -> Mux12/6  "Uy"

== system RobustFormationControl_IntegerModel/Integer Leader and four followers/Follower 1 System/Desired Values ==
  t : Inport
  Helical Trajectry : Subsystem  Commented=on
  Helical Trajectry1 : Subsystem
  Step : Step  Time=0  After=0.001  SampleTime=0
  Step Inputs Trajectry : Subsystem  Commented=on
  Phi_d : Outport  VectorParamsAs1DForOutWhenUnconnected=off
  Theta_d : Outport  Port=2  VectorParamsAs1DForOutWhenUnconnected=off
  Psi_d : Outport  Port=3  VectorParamsAs1DForOutWhenUnconnected=off
  Xd : Outport  Port=4  VectorParamsAs1DForOutWhenUnconnected=off
  Yd : Outport  Port=5  VectorParamsAs1DForOutWhenUnconnected=off
  Zd : Outport  Port=6  VectorParamsAs1DForOutWhenUnconnected=off
  wires:
  t/1 -> Helical Trajectry1/1(t), Helical Trajectry/1(t)
  Step/1 -> Theta_d/1, Phi_d/1
  Helical Trajectry1/1(xd) -> Xd/1
  Helical Trajectry1/4(Psi_d) -> Psi_d/1
  Helical Trajectry1/2(yd) -> Yd/1
  Helical Trajectry1/3(zd) -> Zd/1

== system RobustFormationControl_IntegerModel/Integer Leader and four followers/Follower 1 System/Follower 1 Quadrotor Model ==
  xd : Inport
  yd : Inport  Port=2
  zd : Inport  Port=3
  Psi_d : Inport  Port=4
  xLeader : Inport  Port=5
  dXYZ : Inport  Port=6
  Control Module1 : Subsystem
  Quadrotor Dynamic System : Subsystem
  X : Outport  VectorParamsAs1DForOutWhenUnconnected=off
  Y : Outport  Port=2  VectorParamsAs1DForOutWhenUnconnected=off
  Z : Outport  Port=3  VectorParamsAs1DForOutWhenUnconnected=off
  Phi : Outport  Port=4  VectorParamsAs1DForOutWhenUnconnected=off
  Theta : Outport  Port=5  VectorParamsAs1DForOutWhenUnconnected=off
  Psi : Outport  Port=6  VectorParamsAs1DForOutWhenUnconnected=off
  U1 : Outport  Port=7  VectorParamsAs1DForOutWhenUnconnected=off
  U2 : Outport  Port=8  VectorParamsAs1DForOutWhenUnconnected=off
  U3 : Outport  Port=9  VectorParamsAs1DForOutWhenUnconnected=off
  U4 : Outport  Port=10  VectorParamsAs1DForOutWhenUnconnected=off
  Ux : Outport  Port=11  VectorParamsAs1DForOutWhenUnconnected=off
  Uy : Outport  Port=12  VectorParamsAs1DForOutWhenUnconnected=off
  wires:
  Control Module1/5(Ux) -> Ux/1, Quadrotor Dynamic System/5(Ux)  "Ux"
  Quadrotor Dynamic System/2(y = x9) -> [x9], Y/1  "Y"
  Quadrotor Dynamic System/6(Psi) -> [x5], Psi/1  "Psi"
  Control Module1/4(U4) -> U4/1, Quadrotor Dynamic System/4(U4)  "U4"
  Quadrotor Dynamic System/3(z = x11) -> [x11], Z/1  "Z"
  Quadrotor Dynamic System/4(Phi) -> [x1], Phi/1  "Phi"
  Quadrotor Dynamic System/5(Theta) -> [x3], Theta/1  "Theta"
  Quadrotor Dynamic System/1(x = x7) -> [x7], X/1  "X"
  Control Module1/6(Uy) -> Uy/1, Quadrotor Dynamic System/6(Uy)  "Uy"
  Control Module1/1(U1) -> Quadrotor Dynamic System/1(U1), U1/1  "U1"
  Control Module1/2(U2) -> Quadrotor Dynamic System/2(U2), U2/1  "U2"
  Control Module1/3(U3) -> U3/1, Quadrotor Dynamic System/3(U3)  "U3"
  Control Module1/7(Omega) -> Quadrotor Dynamic System/7(Omega)
  Quadrotor Dynamic System/7(x2) -> [x2]
  Quadrotor Dynamic System/12(zdot = x12) -> [x12]
  Quadrotor Dynamic System/11(ydot = x10) -> [x10]
  Quadrotor Dynamic System/10(xdot = x8) -> [x8]
  Quadrotor Dynamic System/9(x6) -> [x6]
  Quadrotor Dynamic System/8(x4) -> [x4]
  [x1] -> Control Module1/1(x1)
  [x2] -> Control Module1/2(x2)
  [x3] -> Control Module1/3(x3)
  [x4] -> Control Module1/4(x4)
  [x5] -> Control Module1/5(x5)
  [x6] -> Control Module1/6(x6)
  [x7] -> Control Module1/7(x7)
  [x8] -> Control Module1/8(x8)
  [x9] -> Control Module1/9(x9)
  [x10] -> Control Module1/10(x10)
  [x11] -> Control Module1/11(x11)
  [x12] -> Control Module1/12(x12)
  xd/1 -> Control Module1/14(" xd")
  yd/1 -> Control Module1/15(yd)
  zd/1 -> Control Module1/16(" zd")
  Psi_d/1 -> Control Module1/13(Psi_d)
  xLeader/1 -> Control Module1/17(xLeader)
  dXYZ/1 -> Control Module1/18(Distance_d)

== system RobustFormationControl_IntegerModel/Integer Leader and four followers/Follower 1 System/Results Plot ==
  note: yL
  xF : Inport
  xL : Inport  Port=2
  Demux : Demux  Outputs=3
  Demux1 : Demux  Outputs=3
  x : Scope  NumInputPorts=2
  y : Scope  NumInputPorts=2
  z : Scope  NumInputPorts=2
  wires:
  xF/1 -> Demux/1
  xL/1 -> Demux1/1
  Demux/1 -> x/1  "xF"
  Demux1/1 -> x/2  "xL"
  Demux/2 -> y/1  "yF"
  Demux1/2 -> y/2
  Demux/3 -> z/1  "zF"
  Demux1/3 -> z/2  "zL"

== system RobustFormationControl_IntegerModel/Integer Leader and four followers/Follower 1 System/ez ==
  note: error analysis for x - position
  note: error analysis for z - position
  note: error analysis for y - position
  e_x : Inport
  e_y : Inport  Port=2
  e_z : Inport  Port=3
  Abs : Abs  SaturateOnIntegerOverflow=off
  Abs1 : Abs  SaturateOnIntegerOverflow=off
  Abs2 : Abs  SaturateOnIntegerOverflow=off
  Clock1 : Clock
  IAE : Display
  IAE1 : Display
  IAE2 : Display
  ISE : Display
  ISE1 : Display
  ISE2 : Display
  ITAE : Display
  ITAE1 : Display
  ITAE2 : Display
  ITSE : Display
  ITSE1 : Display
  ITSE2 : Display
  Integrator{,1..11} (12 alike) : Integrator
  Math Function : Math  Operator=square
  Math Function1 : Math  Operator=square
  Math Function2 : Math  Operator=square
  Mux : Mux
  Mux1 : Mux
  Mux2 : Mux
  Product{,1..5} (6 alike) : Product
  To Workspace : ToWorkspace  VariableName=Ex1  SampleTime=-1
  To Workspace1 : ToWorkspace  VariableName=Ez1  SampleTime=-1
  To Workspace2 : ToWorkspace  VariableName=Ey1  SampleTime=-1
  wires:
  Abs/1 -> Product/1, Integrator/1
  Integrator/1 -> Mux/1, IAE/1
  Math Function/1 -> Product1/1, Integrator1/1
  Integrator1/1 -> Mux/2, ISE/1
  Product/1 -> Integrator2/1
  Integrator2/1 -> Mux/3, ITAE/1
  Product1/1 -> Integrator3/1
  Integrator3/1 -> Mux/4, ITSE/1
  [time] -> Product1/2, Product/2
  [time] -> Product2/2, Product3/2
  Integrator7/1 -> Mux2/4, ITSE1/1
  Product3/1 -> Integrator7/1
  Integrator6/1 -> Mux2/3, ITAE1/1
  Product2/1 -> Integrator6/1
  Integrator5/1 -> Mux2/2, ISE1/1
  Math Function1/1 -> Integrator5/1, Product3/1
  Integrator4/1 -> Mux2/1, IAE1/1
  Abs1/1 -> Integrator4/1, Product2/1
  [ey] -> Abs1/1, Math Function1/1
  [ez] -> Math Function2/1, Abs2/1
  Abs2/1 -> Product4/1, Integrator8/1
  Integrator8/1 -> Mux1/1, IAE2/1
  Math Function2/1 -> Product5/1, Integrator9/1
  Integrator9/1 -> Mux1/2, ISE2/1
  Product4/1 -> Integrator10/1
  Integrator10/1 -> Mux1/3, ITAE2/1
  Product5/1 -> Integrator11/1
  Integrator11/1 -> Mux1/4, ITSE2/1
  [time] -> Product5/2, Product4/2
  e_x/1 -> [ex]
  e_y/1 -> [ey]
  e_z/1 -> [ez]
  Clock1/1 -> [time]
  [ex] -> Math Function/1, Abs/1
  Mux/1 -> To Workspace/1
  Mux1/1 -> To Workspace1/1
  Mux2/1 -> To Workspace2/1

== system RobustFormationControl_IntegerModel/Integer Leader and four followers/Follower 2 System/Desired Values ==
  t : Inport
  Helical Trajectry : Subsystem  Commented=on
  Helical Trajectry1 : Subsystem
  Step : Step  Time=0  After=0.001  SampleTime=0
  Step Inputs Trajectry : Subsystem  Commented=on
  Phi_d : Outport  VectorParamsAs1DForOutWhenUnconnected=off
  Theta_d : Outport  Port=2  VectorParamsAs1DForOutWhenUnconnected=off
  Psi_d : Outport  Port=3  VectorParamsAs1DForOutWhenUnconnected=off
  Xd : Outport  Port=4  VectorParamsAs1DForOutWhenUnconnected=off
  Yd : Outport  Port=5  VectorParamsAs1DForOutWhenUnconnected=off
  Zd : Outport  Port=6  VectorParamsAs1DForOutWhenUnconnected=off
  wires:
  t/1 -> Helical Trajectry1/1(t), Helical Trajectry/1(t)
  Step/1 -> Theta_d/1, Phi_d/1
  Helical Trajectry1/1(xd) -> Xd/1
  Helical Trajectry1/4(Psi_d) -> Psi_d/1
  Helical Trajectry1/2(yd) -> Yd/1
  Helical Trajectry1/3(zd) -> Zd/1

== system RobustFormationControl_IntegerModel/Integer Leader and four followers/Follower 2 System/Follower 2 Quadrotor Model ==
  xd : Inport
  yd : Inport  Port=2
  zd : Inport  Port=3
  Psi_d : Inport  Port=4
  xLeader : Inport  Port=5
  dXYZ : Inport  Port=6
  Control Module1 : Subsystem
  Quadrotor Dynamic System : Subsystem
  X : Outport  VectorParamsAs1DForOutWhenUnconnected=off
  Y : Outport  Port=2  VectorParamsAs1DForOutWhenUnconnected=off
  Z : Outport  Port=3  VectorParamsAs1DForOutWhenUnconnected=off
  Phi : Outport  Port=4  VectorParamsAs1DForOutWhenUnconnected=off
  Theta : Outport  Port=5  VectorParamsAs1DForOutWhenUnconnected=off
  Psi : Outport  Port=6  VectorParamsAs1DForOutWhenUnconnected=off
  U1 : Outport  Port=7  VectorParamsAs1DForOutWhenUnconnected=off
  U2 : Outport  Port=8  VectorParamsAs1DForOutWhenUnconnected=off
  U3 : Outport  Port=9  VectorParamsAs1DForOutWhenUnconnected=off
  U4 : Outport  Port=10  VectorParamsAs1DForOutWhenUnconnected=off
  Ux : Outport  Port=11  VectorParamsAs1DForOutWhenUnconnected=off
  Uy : Outport  Port=12  VectorParamsAs1DForOutWhenUnconnected=off
  wires:
  Control Module1/5(Ux) -> Ux/1, Quadrotor Dynamic System/5(Ux)  "Ux"
  Quadrotor Dynamic System/2(y = x9) -> [x9], Y/1  "Y"
  Quadrotor Dynamic System/6(Psi) -> [x5], Psi/1  "Psi"
  Control Module1/4(U4) -> U4/1, Quadrotor Dynamic System/4(U4)  "U4"
  Quadrotor Dynamic System/3(z = x11) -> [x11], Z/1  "Z"
  Quadrotor Dynamic System/4(Phi) -> [x1], Phi/1  "Phi"
  Quadrotor Dynamic System/5(Theta) -> [x3], Theta/1  "Theta"
  Quadrotor Dynamic System/1(x = x7) -> [x7], X/1  "X"
  Control Module1/6(Uy) -> Uy/1, Quadrotor Dynamic System/6(Uy)  "Uy"
  Control Module1/1(U1) -> Quadrotor Dynamic System/1(U1), U1/1  "U1"
  Control Module1/2(U2) -> Quadrotor Dynamic System/2(U2), U2/1  "U2"
  Control Module1/3(U3) -> U3/1, Quadrotor Dynamic System/3(U3)  "U3"
  Control Module1/7(Omega) -> Quadrotor Dynamic System/7(Omega)
  Quadrotor Dynamic System/7(x2) -> [x2]
  Quadrotor Dynamic System/12(zdot = x12) -> [x12]
  Quadrotor Dynamic System/11(ydot = x10) -> [x10]
  Quadrotor Dynamic System/10(xdot = x8) -> [x8]
  Quadrotor Dynamic System/9(x6) -> [x6]
  Quadrotor Dynamic System/8(x4) -> [x4]
  [x1] -> Control Module1/1(x1)
  [x2] -> Control Module1/2(x2)
  [x3] -> Control Module1/3(x3)
  [x4] -> Control Module1/4(x4)
  [x5] -> Control Module1/5(x5)
  [x6] -> Control Module1/6(x6)
  [x7] -> Control Module1/7(x7)
  [x8] -> Control Module1/8(x8)
  [x9] -> Control Module1/9(x9)
  [x10] -> Control Module1/10(x10)
  [x11] -> Control Module1/11(x11)
  [x12] -> Control Module1/12(x12)
  xd/1 -> Control Module1/14(" xd")
  yd/1 -> Control Module1/15(yd)
  zd/1 -> Control Module1/16(" zd")
  Psi_d/1 -> Control Module1/13(Psi_d)
  xLeader/1 -> Control Module1/17(xLeader)
  dXYZ/1 -> Control Module1/18(Distance_d)

== system RobustFormationControl_IntegerModel/Integer Leader and four followers/Follower 2 System/Results Plot ==
  note: yL
  xF : Inport
  xL : Inport  Port=2
  Demux : Demux  Outputs=3
  Demux1 : Demux  Outputs=3
  x : Scope  NumInputPorts=2
  y : Scope  NumInputPorts=2
  z : Scope  NumInputPorts=2
  wires:
  xF/1 -> Demux/1
  xL/1 -> Demux1/1
  Demux/1 -> x/1  "xF"
  Demux1/1 -> x/2  "xL"
  Demux/2 -> y/1  "yF"
  Demux1/2 -> y/2
  Demux/3 -> z/1  "zF"
  Demux1/3 -> z/2  "zL"

== system RobustFormationControl_IntegerModel/Integer Leader and four followers/Follower 2 System/ez ==
  note: error analysis for x - position
  note: error analysis for z - position
  note: error analysis for y - position
  e_x : Inport
  e_y : Inport  Port=2
  e_z : Inport  Port=3
  Abs : Abs  SaturateOnIntegerOverflow=off
  Abs1 : Abs  SaturateOnIntegerOverflow=off
  Abs2 : Abs  SaturateOnIntegerOverflow=off
  Clock1 : Clock
  IAE : Display
  IAE1 : Display
  IAE2 : Display
  ISE : Display
  ISE1 : Display
  ISE2 : Display
  ITAE : Display
  ITAE1 : Display
  ITAE2 : Display
  ITSE : Display
  ITSE1 : Display
  ITSE2 : Display
  Integrator{,1..11} (12 alike) : Integrator
  Math Function : Math  Operator=square
  Math Function1 : Math  Operator=square
  Math Function2 : Math  Operator=square
  Mux : Mux
  Mux1 : Mux
  Mux2 : Mux
  Product{,1..5} (6 alike) : Product
  To Workspace : ToWorkspace  VariableName=Ex2  SampleTime=-1
  To Workspace1 : ToWorkspace  VariableName=Ez2  SampleTime=-1
  To Workspace2 : ToWorkspace  VariableName=Ey2  SampleTime=-1
  wires:
  Abs/1 -> Product/1, Integrator/1
  Integrator/1 -> Mux/1, IAE/1
  Math Function/1 -> Product1/1, Integrator1/1
  Integrator1/1 -> Mux/2, ISE/1
  Product/1 -> Integrator2/1
  Integrator2/1 -> Mux/3, ITAE/1
  Product1/1 -> Integrator3/1
  Integrator3/1 -> Mux/4, ITSE/1
  [time] -> Product1/2, Product/2
  [time] -> Product2/2, Product3/2
  Integrator7/1 -> Mux2/4, ITSE1/1
  Product3/1 -> Integrator7/1
  Integrator6/1 -> Mux2/3, ITAE1/1
  Product2/1 -> Integrator6/1
  Integrator5/1 -> Mux2/2, ISE1/1
  Math Function1/1 -> Integrator5/1, Product3/1
  Integrator4/1 -> Mux2/1, IAE1/1
  Abs1/1 -> Integrator4/1, Product2/1
  [ey] -> Abs1/1, Math Function1/1
  [ez] -> Math Function2/1, Abs2/1
  Abs2/1 -> Product4/1, Integrator8/1
  Integrator8/1 -> Mux1/1, IAE2/1
  Math Function2/1 -> Product5/1, Integrator9/1
  Integrator9/1 -> Mux1/2, ISE2/1
  Product4/1 -> Integrator10/1
  Integrator10/1 -> Mux1/3, ITAE2/1
  Product5/1 -> Integrator11/1
  Integrator11/1 -> Mux1/4, ITSE2/1
  [time] -> Product5/2, Product4/2
  e_x/1 -> [ex]
  e_y/1 -> [ey]
  e_z/1 -> [ez]
  Clock1/1 -> [time]
  [ex] -> Math Function/1, Abs/1
  Mux/1 -> To Workspace/1
  Mux1/1 -> To Workspace1/1
  Mux2/1 -> To Workspace2/1

== system RobustFormationControl_IntegerModel/Integer Leader and four followers/Follower 3 System/Desired Values ==
  t : Inport
  Helical Trajectry : Subsystem  Commented=on
  Helical Trajectry1 : Subsystem
  Step : Step  Time=0  After=0.001  SampleTime=0
  Step Inputs Trajectry : Subsystem  Commented=on
  Phi_d : Outport  VectorParamsAs1DForOutWhenUnconnected=off
  Theta_d : Outport  Port=2  VectorParamsAs1DForOutWhenUnconnected=off
  Psi_d : Outport  Port=3  VectorParamsAs1DForOutWhenUnconnected=off
  Xd : Outport  Port=4  VectorParamsAs1DForOutWhenUnconnected=off
  Yd : Outport  Port=5  VectorParamsAs1DForOutWhenUnconnected=off
  Zd : Outport  Port=6  VectorParamsAs1DForOutWhenUnconnected=off
  wires:
  Helical Trajectry1/3(zd) -> Zd/1
  Helical Trajectry1/2(yd) -> Yd/1
  Helical Trajectry1/4(Psi_d) -> Psi_d/1
  Helical Trajectry1/1(xd) -> Xd/1
  Step/1 -> Phi_d/1, Theta_d/1
  t/1 -> Helical Trajectry/1(t), Helical Trajectry1/1(t)

== system RobustFormationControl_IntegerModel/Integer Leader and four followers/Follower 3 System/Follower 2 Quadrotor Model ==
  xd : Inport
  yd : Inport  Port=2
  zd : Inport  Port=3
  Psi_d : Inport  Port=4
  xLeader : Inport  Port=5
  dXYZ : Inport  Port=6
  Control Module1 : Subsystem
  Quadrotor Dynamic System : Subsystem
  X : Outport  VectorParamsAs1DForOutWhenUnconnected=off
  Y : Outport  Port=2  VectorParamsAs1DForOutWhenUnconnected=off
  Z : Outport  Port=3  VectorParamsAs1DForOutWhenUnconnected=off
  Phi : Outport  Port=4  VectorParamsAs1DForOutWhenUnconnected=off
  Theta : Outport  Port=5  VectorParamsAs1DForOutWhenUnconnected=off
  Psi : Outport  Port=6  VectorParamsAs1DForOutWhenUnconnected=off
  U1 : Outport  Port=7  VectorParamsAs1DForOutWhenUnconnected=off
  U2 : Outport  Port=8  VectorParamsAs1DForOutWhenUnconnected=off
  U3 : Outport  Port=9  VectorParamsAs1DForOutWhenUnconnected=off
  U4 : Outport  Port=10  VectorParamsAs1DForOutWhenUnconnected=off
  Ux : Outport  Port=11  VectorParamsAs1DForOutWhenUnconnected=off
  Uy : Outport  Port=12  VectorParamsAs1DForOutWhenUnconnected=off
  wires:
  dXYZ/1 -> Control Module1/18(Distance_d)
  xLeader/1 -> Control Module1/17(xLeader)
  Psi_d/1 -> Control Module1/13(Psi_d)
  zd/1 -> Control Module1/16(" zd")
  yd/1 -> Control Module1/15(yd)
  xd/1 -> Control Module1/14(" xd")
  [x12] -> Control Module1/12(x12)
  [x11] -> Control Module1/11(x11)
  [x10] -> Control Module1/10(x10)
  [x9] -> Control Module1/9(x9)
  [x8] -> Control Module1/8(x8)
  [x7] -> Control Module1/7(x7)
  [x6] -> Control Module1/6(x6)
  [x5] -> Control Module1/5(x5)
  [x4] -> Control Module1/4(x4)
  [x3] -> Control Module1/3(x3)
  [x2] -> Control Module1/2(x2)
  [x1] -> Control Module1/1(x1)
  Quadrotor Dynamic System/8(x4) -> [x4]
  Quadrotor Dynamic System/9(x6) -> [x6]
  Quadrotor Dynamic System/10(xdot = x8) -> [x8]
  Quadrotor Dynamic System/11(ydot = x10) -> [x10]
  Quadrotor Dynamic System/12(zdot = x12) -> [x12]
  Quadrotor Dynamic System/7(x2) -> [x2]
  Control Module1/7(Omega) -> Quadrotor Dynamic System/7(Omega)
  Control Module1/3(U3) -> Quadrotor Dynamic System/3(U3), U3/1  "U3"
  Control Module1/2(U2) -> U2/1, Quadrotor Dynamic System/2(U2)  "U2"
  Control Module1/1(U1) -> U1/1, Quadrotor Dynamic System/1(U1)  "U1"
  Control Module1/6(Uy) -> Quadrotor Dynamic System/6(Uy), Uy/1  "Uy"
  Quadrotor Dynamic System/1(x = x7) -> X/1, [x7]  "X"
  Quadrotor Dynamic System/5(Theta) -> Theta/1, [x3]  "Theta"
  Quadrotor Dynamic System/4(Phi) -> Phi/1, [x1]  "Phi"
  Quadrotor Dynamic System/3(z = x11) -> Z/1, [x11]  "Z"
  Control Module1/4(U4) -> Quadrotor Dynamic System/4(U4), U4/1  "U4"
  Quadrotor Dynamic System/6(Psi) -> Psi/1, [x5]  "Psi"
  Quadrotor Dynamic System/2(y = x9) -> Y/1, [x9]  "Y"
  Control Module1/5(Ux) -> Quadrotor Dynamic System/5(Ux), Ux/1  "Ux"

== system RobustFormationControl_IntegerModel/Integer Leader and four followers/Follower 3 System/Results Plot ==
  note: yL
  xF : Inport
  xL : Inport  Port=2
  Demux : Demux  Outputs=3
  Demux1 : Demux  Outputs=3
  x : Scope  NumInputPorts=2
  y : Scope  NumInputPorts=2
  z : Scope  NumInputPorts=2
  wires:
  Demux1/3 -> z/2  "zL"
  Demux/3 -> z/1  "zF"
  Demux1/2 -> y/2
  Demux/2 -> y/1  "yF"
  Demux1/1 -> x/2  "xL"
  Demux/1 -> x/1  "xF"
  xL/1 -> Demux1/1
  xF/1 -> Demux/1
